simulink model "ControlLogic"  (R2025a)
settings: Solver=ode3  StartTime=0.0  StopTime=20  FixedStep=0.001  MaxStep=1e-4  RelTol=1e-3  EnableMultiTasking=on
Description:
  | Copyright 2016-2025 The MathWorks, Inc.
settings Model: MinMaxOverflowLogging=ForceOff  Creator=smiller  LastModifiedBy=smiller
settings SolverCC: AlgebraicLoopSolver=TrustRegion
settings DataIOCC: LimitDataPoints=on  SaveFormat=StructureWithTime  SignalLoggingSaveFormat=ModelDataLogs  SaveOutput=off  SaveTime=off  ReturnWorkspaceOutputs=off
settings OptimizationCC: ReuseModelBlockBuffer=off  ExpressionDepthLimit=2147483647.0  LifeSpan=inf
settings DebuggingCC: UnderspecifiedInitializationDetection=Classic  MergeDetectMultiDrivingBlocksExec=none  InheritedTsInSrcMsg=none  FcnCallInpInsideContextMsg=warning  UnconnectedInputMsg=warning  UnconnectedOutputMsg=warning  UnconnectedLineMsg=warning  BusObjectLabelMismatch=error  AllowSymbolicDim=off  StateNameClashWarn=warning  PregeneratedLibrarySubsystemCodeDiagnostic=none  SFUnexpectedBacktrackingDiag=warning  SFNoUnconditionalDefaultTransitionDiag=warning  SFExecutionAtInitializationDiag=none  ArithmeticOperatorsInVariantConditions=warning
settings HardwareCC: ProdBitPerPointer=32.0  ProdBitPerSizeT=32.0  ProdBitPerPtrDiffT=32.0  ProdLargestAtomicFloat=None  ProdIntDivRoundTo=Undefined  ProdEndianess=Unspecified  ProdWordSize=32.0  ProdHWDeviceType=32-bit Generic
settings ModelReferenceCC: UpdateModelReferenceTargets=IfOutOfDate  EnableRefExpFcnMdlSchedulingChecks=on  PropagateSignalLabelsOutOfModel=off
settings SFSimCC: SimUseLocalCustomCode=off  SimParseCustomCode=off  CustomCodeUndefinedFunction=UseInterfaceOnly
settings RTWCC: RTWUseLocalCustomCode=off  GPUComputeCapability=3.5  DLArmComputeVersion=19.05
settings CodeAppCC: StateflowObjectComments=on
settings GRTTargetCC: TargetLangStandard=C89/C90 (ANSI)  CombineOutputUpdateFcns=off  GRTInterface=on
settings ConfigComp: CovEnable=on  CovScope=Subsystem  RecordCoverage=on  CovPath=Turbine State Machine  CovMetricSettings=dcm  CovHTMLOptions=-sRT=1 -sVT=1 -aTS=1 -bRG=1 -bTC=1 -hTR=0 -nFC=0 -scm=1 -bcm=1 -xEv=0  CovForceBlockReductionOff=off  CovSaveCumulativeToWorkspaceVar=on  CovCumulativeVarName=covCumulativeData_JBR  CovExternalEMLEnable=off  CovSFcnEnable=off  DVMaxProcessTime=300.0  DVModelCoverageObjectives=MCDC  DVMaxTestCaseSteps=500.0  DVTestSuiteOptimization=Auto  DVIgnoreCovSatisfied=on  DVCoverageDataFile=covCumulativeData_JBR.cvt  DVAbsoluteTolerance=1.0e-5  DVDefectChecker=off  DVDetectDeadLogic=on  DVMaxViolationSteps=20.0  DVHarnessSource=Signal Editor  DVSaveReport=on  DVDisplayResultsOnModel=on  DVRebuildModelRepresentation=Always  DVActiveTab=0.0

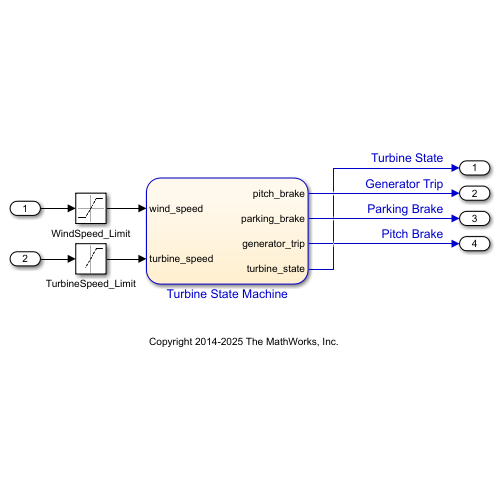
[thumbnail: Simulink's stored preview of the top-level diagram]
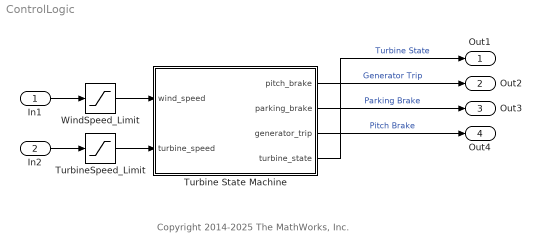
== system ControlLogic ==
  note: Copyright 2014-2025 The MathWorks, Inc.
  In1 : Inport  OutDataTypeStr=double  PortDimensions=1  SampleTime=0.001
  In2 : Inport  Port=2  OutDataTypeStr=double  PortDimensions=1  SampleTime=0.001
  Turbine State Machine : Stateflow chart  TreatAsAtomicUnit=on
  TurbineSpeed_Limit : Saturate  UpperLimit=2500  LowerLimit=0
  WindSpeed_Limit : Saturate  UpperLimit=50  LowerLimit=0
  Out1 : Outport  OutDataTypeStr=double  PortDimensions=1  SampleTime=[0.001,0]  VectorParamsAs1DForOutWhenUnconnected=off
  Out2 : Outport  Port=2  OutDataTypeStr=double  PortDimensions=1  SampleTime=[0.001,0]  VectorParamsAs1DForOutWhenUnconnected=off
  Out3 : Outport  Port=3  OutDataTypeStr=double  PortDimensions=1  SampleTime=[0.001,0]  VectorParamsAs1DForOutWhenUnconnected=off
  Out4 : Outport  Port=4  OutDataTypeStr=double  PortDimensions=1  SampleTime=[0.001,0]  VectorParamsAs1DForOutWhenUnconnected=off
  wires:
  Turbine State Machine/3(generator_trip) -> Out4/1  "Pitch Brake"
  Turbine State Machine/2(parking_brake) -> Out3/1  "Parking Brake"
  Turbine State Machine/1(pitch_brake) -> Out2/1  "Generator Trip"
  Turbine State Machine/4(turbine_state) -> Out1/1  "Turbine State"
  In1/1 -> WindSpeed_Limit/1
  WindSpeed_Limit/1 -> Turbine State Machine/1(wind_speed)
  In2/1 -> TurbineSpeed_Limit/1
  TurbineSpeed_Limit/1 -> Turbine State Machine/2(turbine_speed)

== stateflow chart ControlLogic/Turbine State Machine ==
  state Normal
    state Generating
      entry: parking_brake = 0;
      generator_trip = 0;
      pitch_brake = 0;
      turbine_state = 2;
    state Startup
      entry: parking_brake = 0;
      generator_trip = 1;
      pitch_brake = 0;
      turbine_state = 1;
    state Park
      entry: parking_brake = 1;
      generator_trip = 1;
      pitch_brake = 1;
      turbine_state = 0;
    state Brake
      entry: parking_brake = 0;
      generator_trip = 1;
      pitch_brake = 1;
      turbine_state = 3;
    Startup -> Generating [order 1] : [turbine_speed>...
        | turbine_speed_cut_in]
    Park -> Startup : [wind_speed>...
        | wind_speed_cut_in_lower...
        | &&wind_speed<...
        | wind_speed_cut_out]
    Startup -> Brake [order 2] : [wind_speed<...
        | wind_speed_cut_in_lower]
    Brake -> Startup [order 2] : [wind_speed<...
        | wind_speed_cut_in_upper...
        | && wind_speed>...
        | wind_speed_cut_in_lower]
    Generating -> Brake : [wind_speed<...
        | wind_speed_cut_in_lower...
        | ||wind_speed>...
        | wind_speed_cut_out...
        | ||turbine_speed>...
        | turbine_speed_cut_out...
        | ||turbine_speed<...
        | turbine_speed_cut_in*0.9]
    Brake -> Park [order 1] : [turbine_speed<=...
        | park_speed]
    (default) -> Park
  state Danger
    entry: parking_brake = 1;
    generator_trip = 1;
    pitch_brake = 1;
    turbine_state = 4;
    count = uint16(0);
    during:
    count = count + uint16(1);
  (default) -> Normal
  Normal -> Danger : [wind_speed>50]
  Danger -> Normal : [wind_speed<=50 && count>9999]
  data: pitch_brake output double; wind_speed input; turbine_speed input; parking_brake output double; generator_trip output double; wind_speed_cut_in_lower local double =WT_Params.Main_Controller.wind_speed_cut_in_lower; turbine_speed_cut_in local double =WT_Params.Main_Controller.turbine_speed_cut_in; turbine_state output double; wind_speed_cut_out local double =WT_Params.Main_Controller.wind_speed_cut_out; wind_speed_cut_in_upper local double =WT_Params.Main_Controller.wind_speed_cut_in_upper; turbine_speed_cut_out local double =WT_Params.Main_Controller.turbine_speed_cut_out; park_speed constant double =WT_Params.Main_Controller.turbine_speed_park; count local uint16
